simulink model "buck_converter_input_filter_design_A01"  (R2025b)
settings: Solver=ode23tb  StartTime=0.0  StopTime=1  RelTol=1e-3
values from neighbouring files (symbols this model uses):
  C = 100e-6    (= 0.0001)    [Z_D_and_Z_N_plots_A01.m]    (also in Z_D_and_Z_N_plots_damping_A01.m; Z_D_and_Z_N_plots_undampedA01.m)
  C_b = 4700e-6    (= 0.0047)    [Z_D_and_Z_N_plots_A01.m]    (also in Z_D_and_Z_N_plots_damping_A01.m; Z_D_and_Z_N_plots_undampedA01.m)
  C_f = 370e-6    (= 0.00037)    [Z_D_and_Z_N_plots_A01.m]    (also in Z_D_and_Z_N_plots_damping_A01.m; Z_D_and_Z_N_plots_undampedA01.m)
  L = 100e-6    (= 0.0001)    [Z_D_and_Z_N_plots_A01.m]    (also in Z_D_and_Z_N_plots_damping_A01.m; Z_D_and_Z_N_plots_undampedA01.m)
  L_f = 430e-6    (= 0.00043)    [Z_D_and_Z_N_plots_A01.m]    (also in Z_D_and_Z_N_plots_damping_A01.m; Z_D_and_Z_N_plots_undampedA01.m)
  R = 3    [Z_D_and_Z_N_plots_A01.m]    (also in Z_D_and_Z_N_plots_damping_A01.m; Z_D_and_Z_N_plots_undampedA01.m)
  R_f = 1    [Z_D_and_Z_N_plots_A01.m]    (also in Z_D_and_Z_N_plots_damping_A01.m; Z_D_and_Z_N_plots_undampedA01.m)
libraries: spsSeriesRLCBranchLib x10, spsCurrentMeasurementLib x4, spsDCVoltageSourceLib x2, spsDiodeLib x2, spsMosfetLib x2, spsVoltageMeasurementLib x2, sps_lib x1
settings Model: Creator=arif  LastModifiedBy=arif

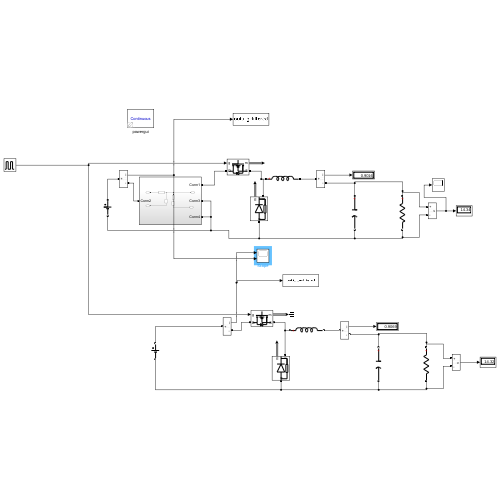
[thumbnail: Simulink's stored preview of the top-level diagram]
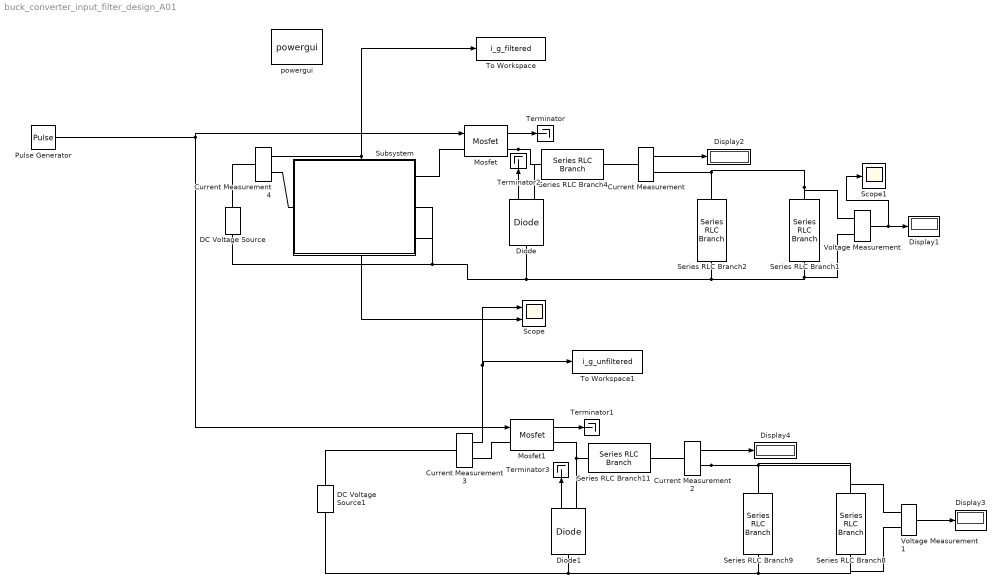
== system buck_converter_input_filter_design_A01 ==
  Current Measurement{,2..4} (4 alike) : spsCurrentMeasurementLib/Current Measurement  PhasorSimulation=off  OutputType=Complex  PSBequivalent=0
  DC Voltage Source : spsDCVoltageSourceLib/DC Voltage Source  Amplitude=30  Measurements=None
  DC Voltage Source1 : spsDCVoltageSourceLib/DC Voltage Source  Amplitude=30  Measurements=None
  Diode : spsDiodeLib/Diode  Ron=0.001  Lon=0  Vf=0.8  IC=0  UseSnubber=0  Rs=500  Cs=250e-9  Measurements=on
  Diode1 : spsDiodeLib/Diode  Ron=0.001  Lon=0  Vf=0.8  IC=0  UseSnubber=0  Rs=500  Cs=250e-9  Measurements=on
  Display{1..4} (4 alike) : Display
  Mosfet : spsMosfetLib/Mosfet  Ron=0.1  Lon=0  Rd=0.01  Vfd=0  IC=0  Rs=1e5  Cs=inf  Measurements=on
  Mosfet1 : spsMosfetLib/Mosfet  Ron=0.1  Lon=0  Rd=0.01  Vfd=0  IC=0  Rs=1e5  Cs=inf  Measurements=on
  Pulse Generator : DiscretePulseGenerator  PulseType=Time based  Period=1/10000  PulseWidth=50
  Scope : Scope  NumInputPorts=2
      settings: ActiveDisplayYMinimum=-2.410247247576339  ActiveDisplayYMaximum=21.692760062419595
  Scope1 : Scope
      settings: ActiveDisplayYMinimum=13.846035187426795  ActiveDisplayYMaximum=14.869005512056839
  Series RLC Branch1 : spsSeriesRLCBranchLib/Series RLC Branch  LConnTagsString=__new0  RConnTagsString=__new0  BranchType=R  Resistance=R  Inductance=1e-3  SetiL0=off  InitialCurrent=0  Capacitance=1e-6  Setx0=off  InitialVoltage=0  Measurements=None
  Series RLC Branch11 : spsSeriesRLCBranchLib/Series RLC Branch  LConnTagsString=__new0  RConnTagsString=__new0  BranchType=L  Resistance=10  Inductance=L  SetiL0=off  InitialCurrent=0  Capacitance=1e-6  Setx0=off  InitialVoltage=0  Measurements=None
  Series RLC Branch2 : spsSeriesRLCBranchLib/Series RLC Branch  LConnTagsString=__new0  RConnTagsString=__new0  BranchType=C  Resistance=10  Inductance=1e-3  SetiL0=off  InitialCurrent=0  Capacitance=C  Setx0=off  InitialVoltage=0  Measurements=None
  Series RLC Branch4 : spsSeriesRLCBranchLib/Series RLC Branch  LConnTagsString=__new0  RConnTagsString=__new0  BranchType=L  Resistance=10  Inductance=L  SetiL0=off  InitialCurrent=0  Capacitance=1e-6  Setx0=off  InitialVoltage=0  Measurements=None
  Series RLC Branch8 : spsSeriesRLCBranchLib/Series RLC Branch  LConnTagsString=__new0  RConnTagsString=__new0  BranchType=R  Resistance=R  Inductance=1e-3  SetiL0=off  InitialCurrent=0  Capacitance=1e-6  Setx0=off  InitialVoltage=0  Measurements=None
  Series RLC Branch9 : spsSeriesRLCBranchLib/Series RLC Branch  LConnTagsString=__new0  RConnTagsString=__new0  BranchType=C  Resistance=10  Inductance=1e-3  SetiL0=off  InitialCurrent=0  Capacitance=C  Setx0=off  InitialVoltage=0  Measurements=None
  Subsystem : Subsystem
  Terminator{,1..3} (4 alike) : Terminator
  To Workspace : ToWorkspace  VariableName=i_g_filtered  SampleTime=-1
  To Workspace1 : ToWorkspace  VariableName=i_g_unfiltered  SampleTime=-1
  Voltage Measurement : spsVoltageMeasurementLib/Voltage Measurement  PhasorSimulation=off  OutputType=Complex  PSBequivalent=0
  Voltage Measurement1 : spsVoltageMeasurementLib/Voltage Measurement  PhasorSimulation=off  OutputType=Complex  PSBequivalent=0
  powergui : sps_lib/powergui  Priority=1  SimulationMode=Continuous  SampleTime=50e-6  frequency=60  Iterations=50  frequencyindice=0  Pbase=100e6  ErrMax=1e-4  UnitsV=kV  UnitsW=MW  buscounter=0  FunctionMessages=off  echomessages=off  EnableUseOfTLC=off  CurrentSourceSwitches=off  DisableSnubberDevices=off  DisableRonSwitches=off  DisableVfSwitches=off  DisplayEquations=off  AutomaticDiscreteSolvers=off  SolverType=Tustin/Backward Euler (TBE)  Interpol=off  ExternalGateDelay=off  methode=off  Ts=100  x0status=blocks  SPID=on  SwTol=0  HookPort=off  NonlinearTolerance=1e-4  nMaxIteration=100  ContinueOnMaxIteration=off  RestoreLinks=warning  ResistiveCurrentMeasurement=off  Frange=[0:2:500]  Ylog=off  Xlog=on  ShowGrid=off  save=off  variable=ZData  structure=0  ZoomFFT=off  StartTime=0.0  cycles=1  DisplayStyle=1  fundamental=60  FreqAxis=off  MaxFrequency=1000  frequencyindicesteady=1  RmsSteady=1  display=off
  wires:
  Current Measurement/1 -> Display2/1
  Diode/1 -> Terminator2/1
  Mosfet/1 -> Terminator/1
  Mosfet1/1 -> Terminator1/1
  Pulse Generator/1 -> Mosfet/1, Mosfet1/1
  Current Measurement3/1 -> Scope/1, To Workspace1/1
  Diode1/1 -> Terminator3/1
  Current Measurement2/1 -> Display4/1
  Voltage Measurement1/1 -> Display3/1
  Current Measurement4/1 -> To Workspace/1, Scope/2
  Voltage Measurement/1 -> Scope1/1, Display1/1
  connections:
  Mosfet/RConn1 -- Diode/RConn1 -- Series RLC Branch4/LConn1
  Voltage Measurement/LConn2 -- DC Voltage Source/LConn1 -- Subsystem/RConn2 -- Subsystem/RConn3 -- Diode/LConn1 -- Series RLC Branch2/RConn1 -- Series RLC Branch1/RConn1
  Series RLC Branch1/LConn1 -- Series RLC Branch2/LConn1 -- Current Measurement/RConn1 -- Voltage Measurement/LConn1
  Current Measurement/LConn1 -- Series RLC Branch4/RConn1
  Diode1/LConn1 -- Voltage Measurement1/LConn2 -- Series RLC Branch8/RConn1 -- Series RLC Branch9/RConn1 -- DC Voltage Source1/LConn1
  Current Measurement2/RConn1 -- Series RLC Branch8/LConn1 -- Voltage Measurement1/LConn1 -- Series RLC Branch9/LConn1
  Series RLC Branch11/LConn1 -- Mosfet1/RConn1 -- Diode1/RConn1
  Current Measurement2/LConn1 -- Series RLC Branch11/RConn1
  Current Measurement3/LConn1 -- DC Voltage Source1/RConn1
  Current Measurement3/RConn1 -- Mosfet1/LConn1
  Current Measurement4/LConn1 -- DC Voltage Source/RConn1
  Subsystem/RConn1 -- Mosfet/LConn1
  Current Measurement4/RConn1 -- Subsystem/LConn1

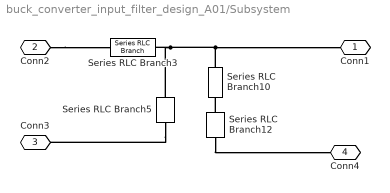
== system buck_converter_input_filter_design_A01/Subsystem ==
  Series RLC Branch10 : spsSeriesRLCBranchLib/Series RLC Branch  LConnTagsString=__new0  RConnTagsString=__new0  BranchType=R  Resistance=R_f  Inductance=1e-3  SetiL0=off  InitialCurrent=0  Capacitance=1e-6  Setx0=off  InitialVoltage=0  Measurements=None
  Series RLC Branch12 : spsSeriesRLCBranchLib/Series RLC Branch  LConnTagsString=__new0  RConnTagsString=__new0  BranchType=C  Resistance=10  Inductance=1e-3  SetiL0=off  InitialCurrent=0  Capacitance=C_b  Setx0=off  InitialVoltage=0  Measurements=None
  Series RLC Branch3 : spsSeriesRLCBranchLib/Series RLC Branch  LConnTagsString=__new0  RConnTagsString=__new0  BranchType=L  Resistance=10  Inductance=L_f  SetiL0=off  InitialCurrent=0  Capacitance=1e-6  Setx0=off  InitialVoltage=0  Measurements=None
  Series RLC Branch5 : spsSeriesRLCBranchLib/Series RLC Branch  LConnTagsString=__new0  RConnTagsString=__new0  BranchType=C  Resistance=10  Inductance=1e-3  SetiL0=off  InitialCurrent=0  Capacitance=C_f  Setx0=off  InitialVoltage=0  Measurements=None
  Conn1 : PMIOPort  Side=Right
  Conn2 : PMIOPort  Port=2  Side=Left
  Conn3 : PMIOPort  Port=3  Side=Right
  Conn4 : PMIOPort  Port=4  Side=Right
  connections:
  Series RLC Branch12/RConn1 -- Conn4/RConn1
  Series RLC Branch12/LConn1 -- Series RLC Branch10/RConn1
  Conn2/RConn1 -- Series RLC Branch3/LConn1
  Series RLC Branch5/LConn1 -- Conn1/RConn1 -- Series RLC Branch10/LConn1 -- Series RLC Branch3/RConn1
  Series RLC Branch5/RConn1 -- Conn3/RConn1
